simulink model "vf_control"  (R2024a)
settings: Solver=ode3  StartTime=0.0  StopTime=11  FixedStep=1e-5  RelTol=1e-3
libraries: spsIGBTDiodeLib x6, simulink x2, spsAsynchronousMachineSIUnitsLib x1, slpidlib x1, spsDCVoltageSourceLib x1, spsGroundLib x1, spsRMSLib x1, spsVoltageMeasurementLib x1, sps_lib x1
settings Model: Creator=LAC060  LastModifiedBy=LAC060
settings DataIOCC: ReturnWorkspaceOutputs=off
settings RTWCC: GPUComputeCapability=3.5

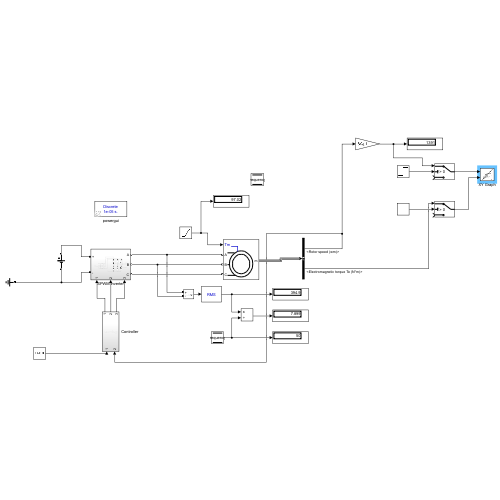
[thumbnail: Simulink's stored preview of the top-level diagram]
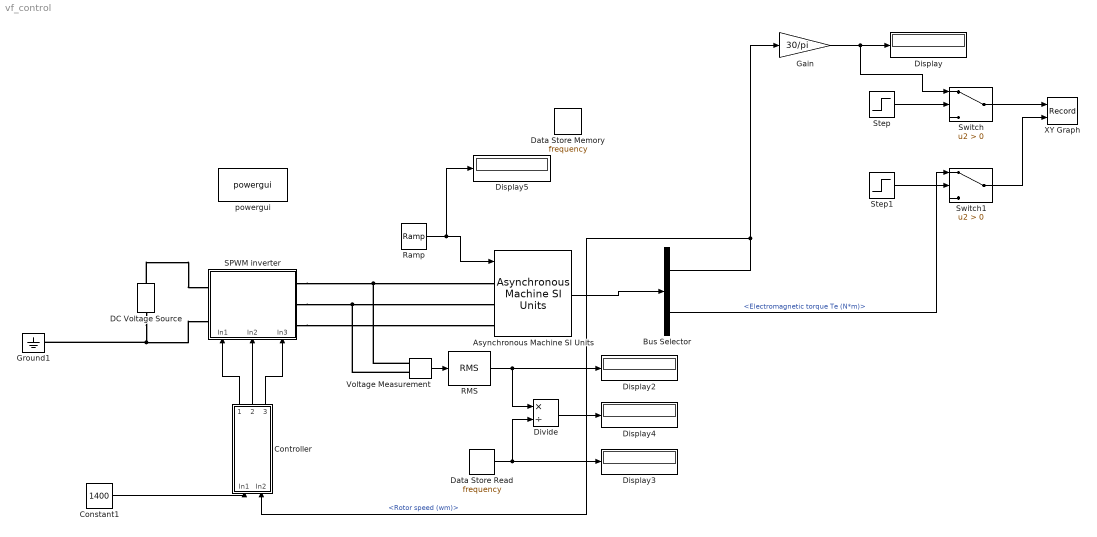
== system vf_control ==
  Asynchronous Machine SI Units : spsAsynchronousMachineSIUnitsLib/Asynchronous Machine SI Units  RotorType=Squirrel-cage  PresetModel=No  MechanicalLoad=Torque Tm  ShowDetailedParameters=on  ReferenceFrame=Rotor  Units=SI  MeasurementBus=off  NominalParameters=[1.845e+04 400 50]  VoltageRatio=1  Stator=[0.5968 0.0003495]  Rotor=[0.6258 0.005473]  Cage1=[0.4155 0.002066]  Cage2=[0.4168 0.0003495]  Lm=0.0354  Mechanical=[0.05 0.005879 2]  PolePairs=2  InitialConditions=[0 0 0 0 0 0 0 0]  SimulateSaturation=off  Saturation=[14.03593122, 27.81365428, 53.79336849, 72.68890987, 97.98006896, 148.6815601, 215.7428561, 302.9841135, 428.7778367 ; 230, 322, 414, 460, 506, 552, 598, 644, 690]  LoadFlowParameters=1492000  TsPowergui=0  TsBlock=-1  IterativeModel=Trapezoidal non iterative  IterativeDiscreteModel=Trapezoidal non iterative  Pmec=1.492e+006
  Bus Selector : BusSelector  OutputSignals=Mechanical.Rotor speed (wm),Mechanical.Electromagnetic torque Te (N*m)
  Constant1 : Constant  Value=1400
  Controller : Subsystem
  DC Voltage Source : spsDCVoltageSourceLib/DC Voltage Source  Amplitude=400*4/sqrt(6)  Measurements=None
  Data Store Memory : DataStoreMemory  DataStoreName=frequency  WriteAfterWriteMsg=warning  ShowAdditionalParam=off
  Data Store Read : DataStoreRead  DataStoreName=frequency  IndexOptions=Index vector (dialog)  Indices=1  OutputSizes=1
  Display{,2..5} (5 alike) : Display
  Divide : Product  Inputs=*/
  Gain : Gain  Gain=30/pi
  Ground1 : spsGroundLib/Ground  LConnTagsString=a
  RMS : spsRMSLib/RMS  TrueRMS=off  Freq=50  RMSInit=120  Ts=0
  Ramp : simulink/Sources/Ramp  slope=10.78  start=2  InitialOutput=0
  SPWM inverter : Subsystem
      settings: PortSchema="{\"entries\":[{\"content\":{\"sides\":[{\"content\":{\"connectorIds\":[\"LConn1\",\"LConn2\"]},\"type\":\"ConnectorPlacement.EquallySpacedRectSide\",\"uuid\":\"53493f46-413b-4a98-8c2d-ae58076bbe31\"},{\"content\":{\"connectorIds\":[\"RConn1\",\"RConn2\",\"RConn3\"],\"side\":\"RIGHT\"},\"type\":\"ConnectorPlacement.EquallySpacedRectSide\",\"uuid\":\"e9d4d61c-066e-46a9-a545-307cf35b1b57\"},{\"content\":{\"side\":\"TOP\"},\"type\":\"ConnectorPlacement.EquallySpacedRectSide\",\"uuid\":\"eb33b145-766b-4ecf-ad8b-1b1d1d9905c1\"},{\"content\":{\"connectorIds\":[\"In1\",\"In2\",\"In3\"],\"side\":\"BOTTOM\"},\"type\":\"ConnectorPlacement.EquallySpacedRectSide\",\"uuid\":\"4c10ecf5-d16f-4d09-b4be-bd4c1e86700b\"}]},\"type\":\"ConnectorPlacement.EquallySpacedConnector\",\"uuid\":\"f174b8e3-9d24-4dfa-9c26-87904651628c\"}],\"packageUris\":[\"http://schema.mathworks.com/mf0/Connector/R2020b\"],\"version\":\"1.0\"}"
  Step : Step  Time=2  SampleTime=0
  Step1 : Step  Time=2  SampleTime=0
  Switch : Switch  Criteria=u2 > Threshold  SaturateOnIntegerOverflow=off  InputSameDT=off
  Switch1 : Switch  Criteria=u2 > Threshold  SaturateOnIntegerOverflow=off  InputSameDT=off
  Voltage Measurement : spsVoltageMeasurementLib/Voltage Measurement  PhasorSimulation=off  OutputType=Complex  PSBequivalent=0
  XY Graph : Record  FileSettingsInternal="{\"entries\":[{\"content\":{\"excelSettings\":{\"content\":{},\"type\":\"Streamout.ExcelSettings\"}},\"type\":\"Streamout.FileSettingStorage\",\"uuid\":\"\"}],\"packageUris\":[\"http:\\/\\/schema.mathworks.com\\/mf0\\/streamout_blocks\\/R2020a\"],\"version\":\"1.0\"}"  Layout=[1 1]  SignalsInternal="{\"entries\":[{\"content\":{\"signals\":[{\"content\":{\"blockPath\":[],\"dimensions\":[1],\"domain\":\"\",\"lineColor\":\"#a2142f\",\"plots\":[ 1 ],\"port\":1,\"sid\":[\"\"],\"signalID\":1,\"signalName\":\"Switch\"},\"type\":\"RecordBlkView.Signal\",\"uuid\":\"\"},{\"content\":{\"blockPath\":[],\"dimensions\":[1],\"domain\":\"\",\"lineColor\":\"#139fff\",\"plots\":[ 1 ],\"port\":2,\"sid\":[\"\"],\"signalID\":2,\"signalName\":\"Switch1\"},\"type\":\"RecordBlkView.Signal\",\"uuid\":\"\"}]},\"type\":\"RecordBlkView.InputSignals\",\"uuid\":\"\"}],\"packageUris\":[\"http:\\/\\/schema.mathworks.com\\/mf0\\/streamout_blocks\\/R2020a\"],\"version\":\"1.0\"}"  VisualizationBindings="{\"xyplotplugin\":{\"info\":[{\"series\":[{\"bindingParametersList\":[{\"parameter\":\"X-Axis\",\"signalID\":1,\"signalName\":\"Switch\"},{\"parameter\":\"Y-Axis\",\"signalID\":2,\"signalName\":\"Switch1\"}],\"seriesID\":0}],\"subplotID\":1}]}}"  CompatibilityTag=XY
  powergui : sps_lib/powergui  Priority=1  SimulationMode=Discrete  SampleTime=1e-5  frequency=60  Iterations=50  frequencyindice=0  Pbase=100e6  ErrMax=1e-4  UnitsV=kV  UnitsW=MW  buscounter=0  FunctionMessages=off  echomessages=off  EnableUseOfTLC=off  CurrentSourceSwitches=off  DisableSnubberDevices=off  DisableRonSwitches=off  DisableVfSwitches=off  DisplayEquations=off  AutomaticDiscreteSolvers=off  SolverType=Tustin  Interpol=off  ExternalGateDelay=off  methode=off  Ts=100  x0status=blocks  SPID=on  SwTol=0  HookPort=off  NonlinearTolerance=1e-4  nMaxIteration=100  ContinueOnMaxIteration=off  RestoreLinks=warning  ResistiveCurrentMeasurement=off  Frange=[0:2:500]  Ylog=off  Xlog=on  ShowGrid=off  save=off  variable=ZData  structure=0  ZoomFFT=off  StartTime=0.0  cycles=1  DisplayStyle=1  fundamental=60  FreqAxis=off  MaxFrequency=1000  frequencyindicesteady=1  RmsSteady=1  display=off
  wires:
  Asynchronous Machine SI Units/1 -> Bus Selector/1
  Ramp/1 -> Display5/1, Asynchronous Machine SI Units/1
  Bus Selector/1 -> Controller/2(In2), Gain/1  "<Rotor speed (wm)>"
  Step/1 -> Switch/2
  Switch/1 -> XY Graph/1
  Step1/1 -> Switch1/2
  Switch1/1 -> XY Graph/2
  Controller/1(Out1) -> SPWM inverter/1(In1)
  Controller/2(Out2) -> SPWM inverter/2(In2)
  Controller/3(Out3) -> SPWM inverter/3(In3)
  Constant1/1 -> Controller/1(In1)
  Gain/1 -> Switch/1, Display/1
  RMS/1 -> Divide/1, Display2/1
  Voltage Measurement/1 -> RMS/1
  Data Store Read/1 -> Divide/2, Display3/1
  Divide/1 -> Display4/1
  Bus Selector/2 -> Switch1/1  "<Electromagnetic torque Te (N*m)>"
  connections:
  DC Voltage Source/RConn1 -- SPWM inverter/LConn1
  DC Voltage Source/LConn1 -- Ground1/LConn1 -- SPWM inverter/LConn2
  SPWM inverter/RConn1 -- Voltage Measurement/LConn1 -- Asynchronous Machine SI Units/LConn1
  SPWM inverter/RConn2 -- Voltage Measurement/LConn2 -- Asynchronous Machine SI Units/LConn2
  SPWM inverter/RConn3 -- Asynchronous Machine SI Units/LConn3

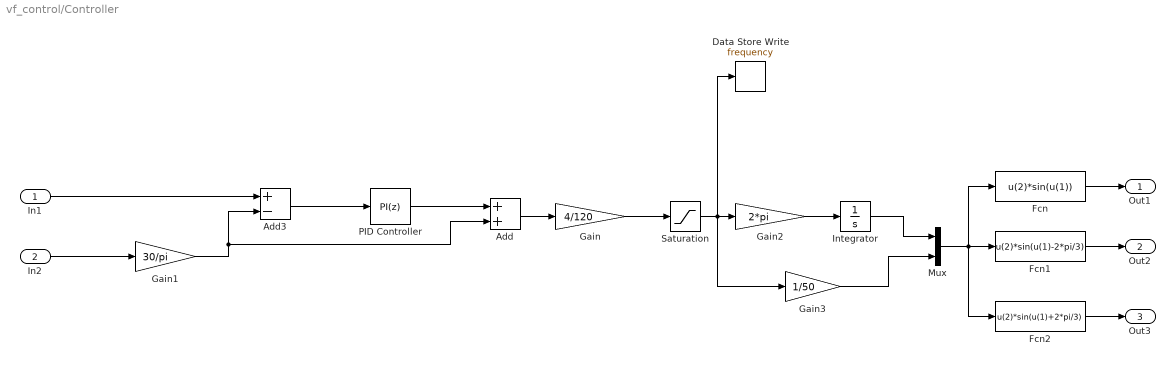
== system vf_control/Controller ==
  In1 : Inport
  In2 : Inport  Port=2
  Add : Sum
  Add3 : Sum  Inputs=+-
  Data Store Write : DataStoreWrite  DataStoreName=frequency  IndexOptions=Index vector (dialog)  Indices=1  OutputSizes=1
  Fcn : Fcn  Expr=u(2)*sin(u(1))
  Fcn1 : Fcn  Expr=u(2)*sin(u(1)-2*pi/3)
  Fcn2 : Fcn  Expr=u(2)*sin(u(1)+2*pi/3)
  Gain : Gain  Gain=4/120
  Gain1 : Gain  Gain=30/pi
  Gain2 : Gain  Gain=2*pi
  Gain3 : Gain  Gain=1/50
  Integrator : Integrator
  Mux : Mux  Inputs=2
  PID Controller : slpidlib/PID Controller  Controller=PI  Form=Parallel  TimeDomain=Discrete-time  UseExternalTs=off  SampleTime=1e-5  IntegratorMethod=Forward Euler  FilterMethod=Forward Euler  ControllerParametersSource=internal  P=1  I=10  UseKiTs=off  D=0  UseExternalDerivativeSource=off  N=100  UseFilter=on  TunerSelectOption=Transfer Function Based (PID Tuner App)  InitialConditionSource=internal  InitialConditionForIntegrator=0  InitialConditionForFilter=0  DifferentiatorICPrevScaledInput=0  ExternalReset=none  TrackingMode=off  Kt=1  LimitOutput=off  SatLimitsSource=internal  UpperSaturationLimit=inf  LowerSaturationLimit=-inf  LinearizeAsGain=on  AntiWindupMode=none  Kb=1  LimitIntegrator=off  UpperIntegratorSaturationLimit=inf  LowerIntegratorSaturationLimit=-inf  POutMin=[]  POutMax=[]  IOutMin=[]  IOutMax=[]  DOutMin=[]  DOutMax=[]  NOutMin=[]  NOutMax=[]  SumOutMin=[]  SumOutMax=[]  SaturationOutMin=[]  SaturationOutMax=[]  PParamMin=[]  PParamMax=[]  IParamMin=[]  IParamMax=[]  DParamMin=[]  DParamMax=[]  NParamMin=[]  NParamMax=[]  KbParamMin=[]  KbParamMax=[]  KtParamMin=[]  KtParamMax=[]  KbOutMin=[]  KbOutMax=[]  KtOutMin=[]  KtOutMax=[]  IntegratorOutMin=[]  IntegratorOutMax=[]  FilterOutMin=[]  FilterOutMax=[]  SumI1OutMin=[]  SumI1OutMax=[]  SumI2OutMin=[]  SumI2OutMax=[]  SumI3OutMin=[]  SumI3OutMax=[]  SumI4OutMin=[]  SumI4OutMax=[]  SumDOutMin=[]  SumDOutMax=[]  DifferentiatorOutMin=[]  DifferentiatorOutMax=[]  FilterDiffOutCoefMin=[]  FilterDiffOutCoefMax=[]  ReciprocalOutMin=[]  ReciprocalOutMax=[]  SumDenOutMin=[]  SumDenOutMax=[]  SumNumOutMin=[]  SumNumOutMax=[]  DivideOutMin=[]  DivideOutMax=[]  UdiffTsProdOutMin=[]  UdiffTsProdOutMax=[]  NTsProdOutMin=[]  NTsProdOutMax=[]  UintegralTsProdOutMin=[]  UintegralTsProdOutMax=[]  UngainTsProdOutMin=[]  UngainTsProdOutMax=[]  ClampingZeroOutDataTypeStr=Inherit: Inherit via back propagation  ClampingZeroOutMin=[]  ClampingZeroOutMax=[]  FilterDenConstantOutDataTypeStr=Inherit: Inherit via back propagation  FilterDenConstantOutMin=[]  FilterDenConstantOutMax=[]  PCopyOutDataTypeStr=Inherit: Inherit via back propagation  PCopyOutMin=[]  PCopyOutMax=[]  NCopyOutDataTypeStr=Inherit: Inherit via back propagation  NCopyOutMin=[]  NCopyOutMax=[]  IntegratorContinuousStateAttributes=''  IntegratorStateMustResolveToSignalObject=off  IntegratorRTWStateStorageClass=Auto  FilterContinuousStateAttributes=''  FilterStateMustResolveToSignalObject=off  FilterRTWStateStorageClass=Auto  ParallelPVariant=InternalParameters  IdealPVariant=Disabled  IVariant=InternalParameters  DVariant=Disabled  IntegratorVariant=Discrete  SatVariant=Disabled  AWVariant=Passthrough  PCopyVariant=Disabled  TRVariant=Disabled  FdbkBlocksVariant=Forward  IdealPFdbkVariant=Disabled  SatFdbkVariant=Disabled  DerivativeFilterVariant=Disabled  NVariant=Disabled  NCopyVariant=Disabled_SignalSpec  FilterICVariant=Disabled  IntegratorICVariant=InternalICs  ExternalResetVariant=Disabled  TRSumVariant=Passthrough  SumFdbkVariant=Disabled  SumVariant=Sum_PI  TsampFilterVariant=InternalTs  TsampNgainVariant=Passthrough  TsampIntegralVariant=Disabled_SignalSpec  ExternalSaturationOutDataTypeStr=Inherit: Same as second input  DerivativeSourceVariant=Disabled
  Saturation : Saturate  UpperLimit=50  LowerLimit=0
  Out1 : Outport
  Out2 : Outport  Port=2
  Out3 : Outport  Port=3
  wires:
  In1/1 -> Add3/1
  Gain1/1 -> Add/2, Add3/2
  Add3/1 -> PID Controller/1
  PID Controller/1 -> Add/1
  Gain/1 -> Saturation/1
  Saturation/1 -> Data Store Write/1, Gain3/1, Gain2/1
  Gain2/1 -> Integrator/1
  Integrator/1 -> Mux/1
  Gain3/1 -> Mux/2
  Mux/1 -> Fcn2/1, Fcn1/1, Fcn/1
  Fcn/1 -> Out1/1
  Fcn1/1 -> Out2/1
  Fcn2/1 -> Out3/1
  In2/1 -> Gain1/1
  Add/1 -> Gain/1

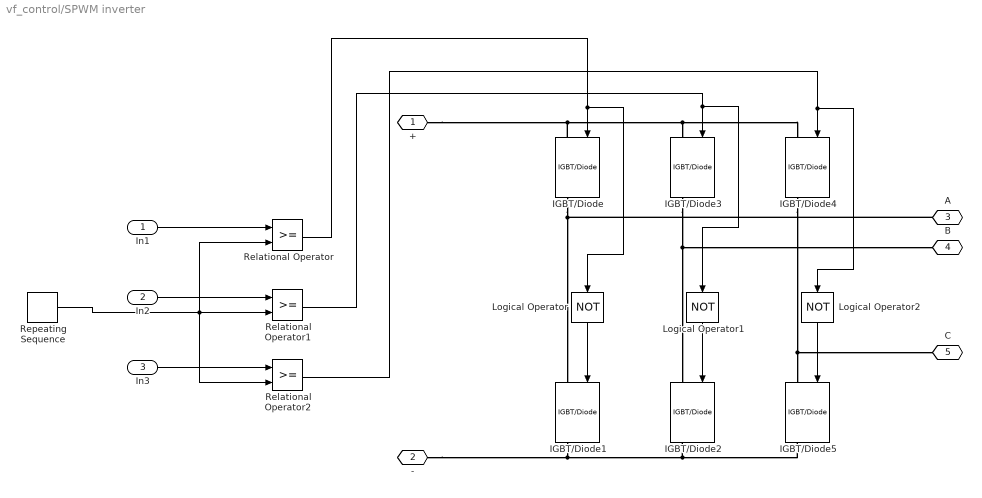
== system vf_control/SPWM inverter ==
  In1 : Inport
  In2 : Inport  Port=2
  In3 : Inport  Port=3
  IGBT/Diode{,1..5} (6 alike) : spsIGBTDiodeLib/IGBT//Diode  Ron=1e-3  Rs=1e5  Cs=inf  Measurements=on
  Logical Operator : Logic  Operator=NOT  AllPortsSameDT=off  OutDataTypeStr=boolean
  Logical Operator1 : Logic  Operator=NOT  AllPortsSameDT=off  OutDataTypeStr=boolean
  Logical Operator2 : Logic  Operator=NOT  AllPortsSameDT=off  OutDataTypeStr=boolean
  Relational Operator : RelationalOperator  OutDataTypeStr=boolean  RndMeth=Simplest  InputSameDT=off
  Relational Operator1 : RelationalOperator  OutDataTypeStr=boolean  RndMeth=Simplest  InputSameDT=off
  Relational Operator2 : RelationalOperator  OutDataTypeStr=boolean  RndMeth=Simplest  InputSameDT=off
  Repeating Sequence : simulink/Sources/Repeating Sequence  rep_seq_t=[0 1 2]/5000  rep_seq_y=[-1 1 -1]
  + : PMIOPort  Side=Left
  - : PMIOPort  Port=2  Side=Left
  A : PMIOPort  Port=3  Side=Right
  B : PMIOPort  Port=4  Side=Right
  C : PMIOPort  Port=5  Side=Right
  wires:
  Repeating Sequence/1 -> Relational Operator/2, Relational Operator2/2, Relational Operator1/2
  In1/1 -> Relational Operator/1
  In2/1 -> Relational Operator1/1
  In3/1 -> Relational Operator2/1
  Logical Operator/1 -> IGBT/Diode1/1
  Logical Operator1/1 -> IGBT/Diode2/1
  Logical Operator2/1 -> IGBT/Diode5/1
  Relational Operator/1 -> Logical Operator/1, IGBT/Diode/1
  Relational Operator1/1 -> Logical Operator1/1, IGBT/Diode3/1
  Relational Operator2/1 -> Logical Operator2/1, IGBT/Diode4/1
  connections:
  IGBT/Diode/RConn1 -- A/RConn1 -- IGBT/Diode1/LConn1
  IGBT/Diode3/RConn1 -- IGBT/Diode2/LConn1 -- B/RConn1
  IGBT/Diode4/RConn1 -- IGBT/Diode5/LConn1 -- C/RConn1
  IGBT/Diode/LConn1 -- +/RConn1 -- IGBT/Diode4/LConn1 -- IGBT/Diode3/LConn1
  IGBT/Diode1/RConn1 -- -/RConn1 -- IGBT/Diode5/RConn1 -- IGBT/Diode2/RConn1
